simulink model "monopile"  (R2021a)
settings: Solver=ode45  StartTime=0  StopTime=10  FixedStep=0.001  MaxStep=0.001  RelTol=1e-3
undefined symbols (not defined in the file or in its folder): body, constraint, geometry, hydroData
libraries: WECSim_Lib_Constraints x2, WECSim_Lib_Body_Elements x2, WECSim_Lib_Frames x1
settings Model: Creator=akeeste  LastModifiedBy=kmruehl
settings SolverCC: ZeroCrossControl=DisableAll  AlgebraicLoopSolver=TrustRegion  AutoInsertRateTranBlk=on
settings DataIOCC: ReturnWorkspaceOutputs=off
settings OptimizationCC: SimCompilerOptimization=on

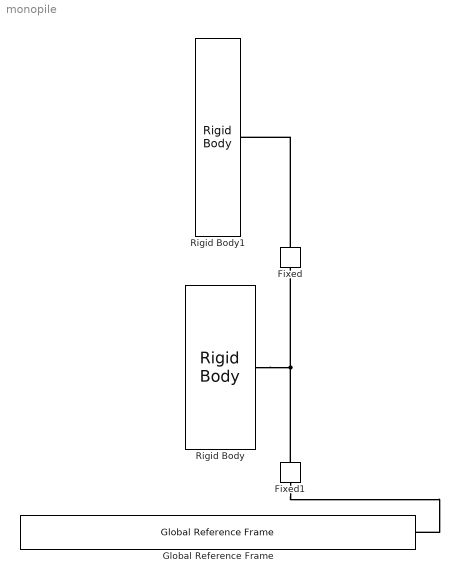
== system monopile ==
  Fixed : WECSim_Lib_Constraints/Fixed  constraint=constraint(2)  loc="0  0  0"  displacement=0 0 0  y=0 1 0  z=0 0 1  upperLimitSpecify=off  upperLimitBound=0  upperLimitTransitionRegionWidth=0  upperLimitStiffness=0  upperLimitDamping=0  lowerLimitSpecify=off  lowerLimitBound=0  lowerLimitTransitionRegionWidth=0  lowerLimitStiffness=0  lowerLimitDamping=0
      settings: AttributesFormatString=%<constraint>  SourceProductName=WEC-Sim
  Fixed1 : WECSim_Lib_Constraints/Fixed  constraint=constraint(1)  loc="0  0  0"  displacement=0 0 0  y=0 1 0  z=0 0 1  upperLimitSpecify=off  upperLimitBound=0  upperLimitTransitionRegionWidth=0  upperLimitStiffness=0  upperLimitDamping=0  lowerLimitSpecify=off  lowerLimitBound=0  lowerLimitTransitionRegionWidth=0  lowerLimitStiffness=0  lowerLimitDamping=0
      settings: AttributesFormatString=%<constraint>  SourceProductName=WEC-Sim
  Global Reference Frame : WECSim_Lib_Frames/Global Reference Frame  waves=waves  simu=simu  InputMethod=Input File  InputFile=wecSimInputFile.m  mode=normal  explorer=off  solver=ode4  startTime=0  rampTime=100  endTime=400  dt=0.1  cicEndTime=60  stateSpace=0  WaveClass=regular  H=2.5  T=8  elevationFile=NOT DEFINED  spectrumFile=NOT DEFINED  direction=0  spread=1  spectrumType=NOT DEFINED  phaseSeed=0  option=EqualEnergy
      settings: SourceProductName=WEC-Sim
  Rigid Body : WECSim_Lib_Body_Elements/Rigid Body  body=body(1)  h5File=hydroData/*.h5  geometryFile=geometry/*.stl  mass=0  momOfInertia=0 0 0  nonHydro=0  nonlinearHydro=0  cg=0 0 0  cb=0 0 0  dof=6  volume=0  displacement=0 0 0  axis=0 1 0  angle=0  option=0  cd=0 0 0  ca=0 0 0  area=0 0 0  VME=0  rgME=0 0 0  z=0 0 1
      settings: SourceProductName=WEC-Sim
  Rigid Body1 : WECSim_Lib_Body_Elements/Rigid Body  body=body(2)  h5File=hydroData/*.h5  geometryFile=geometry/*.stl  mass=0  momOfInertia=0 0 0  nonHydro=0  nonlinearHydro=0  cg=0 0 0  cb=0 0 0  dof=6  volume=0  displacement=0 0 0  axis=0 1 0  angle=0  option=0  cd=0 0 0  ca=0 0 0  area=0 0 0  VME=0  rgME=0 0 0  z=0 0 1
      settings: SourceProductName=WEC-Sim
  connections:
  Fixed1/LConn1 -- Global Reference Frame/RConn1
  Fixed/RConn1 -- Rigid Body1/RConn1
  Rigid Body/RConn1 -- Fixed/LConn1 -- Fixed1/RConn1
